simulink model "test_online"  (R2024b)
settings: Solver=FixedStepAuto  StartTime=0.0  StopTime=inf  FixedStep=0.005  RelTol=1e-3
libraries: androidsensorlib x2, deeplib x1, androidaudiovideolib x1
settings Model: Creator=alessandro  LastModifiedBy=marta
settings OptimizationCC: DefaultParameterBehavior=Inlined  EnhancedBackFolding=on  PassReuseOutputArgsAs=Individual arguments  ZeroExternalMemoryAtStartup=off  ZeroInternalMemoryAtStartup=off  MaxStackSize=64  OptimizeBlockOrder=speed  DifferentSizesBufferReuse=on  OptimizationCustomize=off  EfficientTunableParamExpr=on
settings DebuggingCC: ParameterTunabilityLossMsg=error
settings HardwareCC: ProdBitPerPointer=32  ProdBitPerSizeT=32  ProdBitPerPtrDiffT=32  ProdLargestAtomicInteger=Long  ProdLargestAtomicFloat=Double  ProdWordSize=32  ProdHWDeviceType=ARM Compatible->ARM Cortex-A (32-bit)  UseEmbeddedCoderFeatures=off  UseSimulinkCoderFeatures=off
settings SFSimCC: MATLABDynamicMemAlloc=off
settings RTWCC: Description=Embedded Coder  SystemTargetFile=ert.tlc  HardwareBoard=Android Device  TLCOptions="-aInlineSetEventsForThisBaseRateFcn=TLC_FALSE -aSuppressMultiTaskScheduler=TLC_FALSE  -aRateBasedStepFcn=0"  TemplateMakefile=ert_default_tmf  RTWVerbose=off  Toolchain=Android SDK/NDK Tools
settings CodeAppCC: ForceParamTrailComments=on  IgnoreCustomStorageClasses=off  OperatorAnnotations=on  SimulinkDataObjDesc=on  SFDataObjDesc=on  MangleLength=10  InsertBlockDesc=on
settings ERTTargetCC: SupportNonInlinedSFcns=on

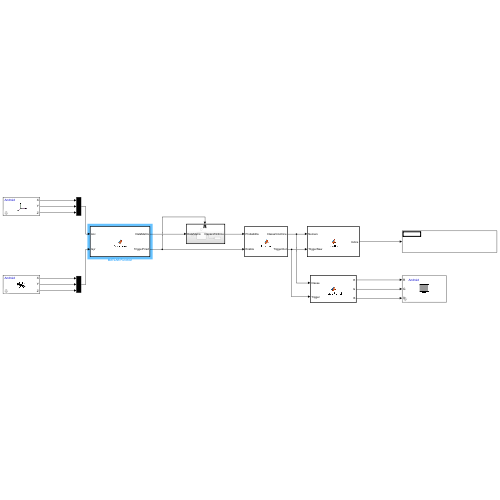
[thumbnail: Simulink's stored preview of the top-level diagram]
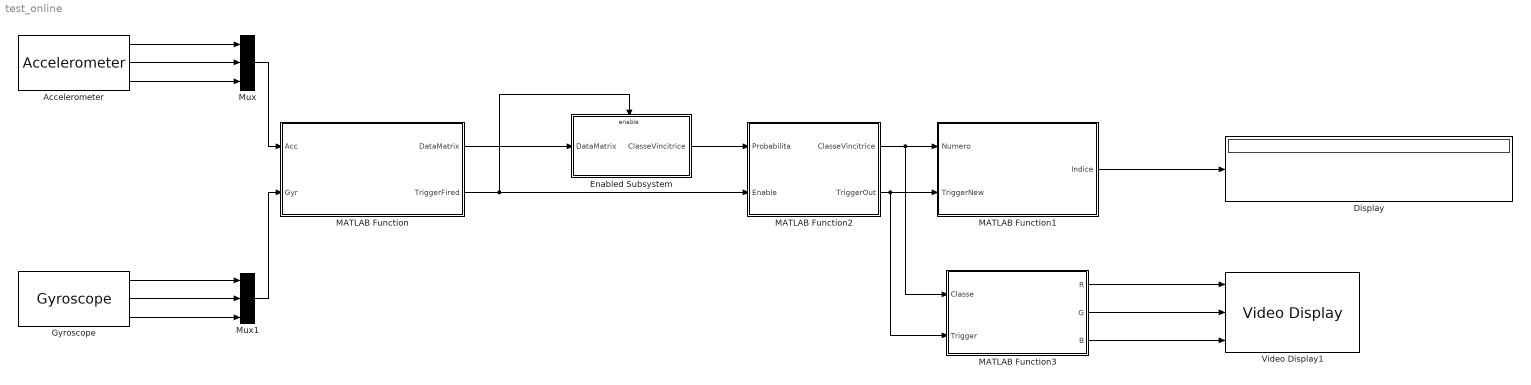
== system test_online ==
  Accelerometer : androidsensorlib/Accelerometer  OutputVector=off  SampleTime=0.005  BlockPlatform=Android
  Display : Display
  Enabled Subsystem : Subsystem  TreatAsAtomicUnit=on
  Gyroscope : androidsensorlib/Gyroscope  OutputVector=off  SampleTime=0.005  BlockPlatform=Android
  MATLAB Function : MATLAB Function  TreatAsAtomicUnit=on
  MATLAB Function1 : MATLAB Function  TreatAsAtomicUnit=on
  MATLAB Function2 : MATLAB Function  TreatAsAtomicUnit=on
  MATLAB Function3 : MATLAB Function  TreatAsAtomicUnit=on
  Mux : Mux  Inputs=3
  Mux1 : Mux  Inputs=3
  Video Display1 : androidaudiovideolib/Video Display  BlockPlatform=Android
  wires:
  MATLAB Function/1(DataMatrix) -> Enabled Subsystem/1(DataMatrix)
  MATLAB Function/2(TriggerFired) -> MATLAB Function2/2(Enable), Enabled Subsystem/Enable
  Accelerometer/1 -> Mux/1
  Accelerometer/2 -> Mux/2
  Accelerometer/3 -> Mux/3
  Mux/1 -> MATLAB Function/1(Acc)
  Gyroscope/1 -> Mux1/1
  Gyroscope/2 -> Mux1/2
  Gyroscope/3 -> Mux1/3
  Mux1/1 -> MATLAB Function/2(Gyr)
  Enabled Subsystem/1(ClasseVincitrice) -> MATLAB Function2/1(Probabilita)
  MATLAB Function2/1(ClasseVincitrice) -> MATLAB Function3/1(Classe), MATLAB Function1/1(Numero)
  MATLAB Function2/2(TriggerOut) -> MATLAB Function1/2(TriggerNew), MATLAB Function3/2(Trigger)
  MATLAB Function1/1(Indice) -> Display/1
  MATLAB Function3/1(R) -> Video Display1/1
  MATLAB Function3/2(G) -> Video Display1/2
  MATLAB Function3/3(B) -> Video Display1/3

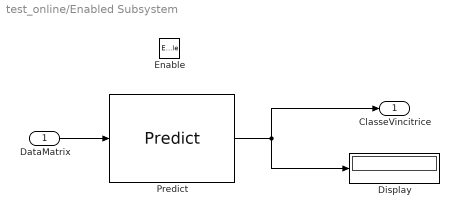
== system test_online/Enabled Subsystem ==
  DataMatrix : Inport
  Enable : EnablePort
  Display : Display
  Predict : deeplib/Predict  Network=Network from MAT-file  NetworkFunction=squeezenet  NetworkFilePath=Rete_CNN_Finale.mat  MiniBatchSize=128  InputDataFormats={ 'input', 'TCB' }  Predictions=on  Activations={}  ForceInterpretedSim=off  EnableDLNetwork=on  LastKnownNetworkFilePath='Rete_CNN_Finale.mat'  LastKnownNetworkTimeStamp=739962.956712962943129241466522216796875
  ClasseVincitrice : Outport
  wires:
  DataMatrix/1 -> Predict/1
  Predict/1 -> Display/1, ClasseVincitrice/1

== matlab function test_online/MATLAB Function ==
  data: Acc input; DataMatrix output; Gyr input; TriggerFired output
function [DataMatrix, TriggerFired] = Processor_Complete(Acc, Gyr)
    Acc = double(Acc(:)).';
    Gyr = double(Gyr(:)).';

    persistent buffer_acc buffer_gyr
    persistent state counter
    persistent baseline_ema
    persistent b_filt a_filt
    persistent z_state          
    persistent startup_timer
    persistent ema_state        

    % --- PARAMETRI ---
    FS = 200;

    WIN_LEN  = 401;
    POST_SEC = 1.0;
    SAMPLES_POST = round(POST_SEC * FS);

    WARMUP_TIME = WIN_LEN;

    % Trigger baseline EMA
    ALPHA_BASELINE = 0.01;
    K_SOGLIA = 2;
    SOGLIA_MIN = 0.1;

    % Smoothing EMA segnale
    ALPHA_SMOOTH = 0.2;

    % --- OUTPUT DEFAULT ---
    TriggerFired = false;
    DataMatrix   = zeros(WIN_LEN, 6, 'single');

    % --- INIZIALIZZAZIONE ---
    if isempty(buffer_acc)
        buffer_acc = zeros(WIN_LEN, 3);
        buffer_gyr = zeros(WIN_LEN, 3);

        state   = 0;
        counter = 0;

        baseline_ema = 0.0;
        startup_timer = WARMUP_TIME;

        [b_filt, a_filt] = butter(2, [0.5 20] / (FS/2), 'bandpass');

        nf = max(length(a_filt), length(b_filt)) - 1;
        z_state = zeros(nf, 6);

        ema_state = zeros(1, 6);
    end

    % --- COSTRUISCI CAMPIONE 1x6 ---
    raw_input = [Acc, Gyr];  % 1x6

    % --- FILTRAGGIO ONLINE CANALE-PER-CANALE ---
    filt_sample = zeros(1, 6);

    for ch = 1:6
        % filtra un campione scalare
        [y, zf] = filter(b_filt, a_filt, raw_input(ch), z_state(:,ch));
        filt_sample(ch) = y;
        z_state(:,ch) = zf;
    end

    % --- SMOOTHING EMA SUI 6 CANALI ---
    ema_state = (1 - ALPHA_SMOOTH) * ema_state + ALPHA_SMOOTH * filt_sample;
    smooth_sample = ema_state;

    Acc_Filt = smooth_sample(1:3);
    Gyr_Filt = smooth_sample(4:6);

    % --- AGGIORNAMENTO BUFFER ---
    buffer_acc = [buffer_acc(2:end, :); Acc_Filt];
    buffer_gyr = [buffer_gyr(2:end, :); Gyr_Filt];

    % --- WARMUP (aggiorna baseline) ---
    acc_y = abs(Acc_Filt(2));

    if startup_timer > 0
        baseline_ema = (1 - ALPHA_BASELINE) * baseline_ema + ALPHA_BASELINE * acc_y;
        startup_timer = startup_timer - 1;
        return;
    end

    % --- SOGLIA ADATTIVA ---
    baseline_ema = (1 - ALPHA_BASELINE) * baseline_ema + ALPHA_BASELINE * acc_y;
    soglia = K_SOGLIA * baseline_ema;
    if soglia < SOGLIA_MIN
        soglia = SOGLIA_MIN;
    end

    % --- MACCHINA A STATI ---
    if state == 0
        if acc_y > soglia
            state = 1;
            counter = 0;
        end

    else % state == 1
        counter = counter + 1;

        if counter >= SAMPLES_POST
            % --- Z-SCORE SU FINESTRA ---
            mu_a  = mean(buffer_acc, 1);
            sig_a = std(buffer_acc, 0, 1);
            mu_g  = mean(buffer_gyr, 1);
            sig_g = std(buffer_gyr, 0, 1);

            sig_a(sig_a == 0) = 1;
            sig_g(sig_g == 0) = 1;

            a_norm = (buffer_acc - mu_a) ./ sig_a;
            g_norm = (buffer_gyr - mu_g) ./ sig_g;

            DataMatrix   = single([a_norm, g_norm]);
            TriggerFired = true;

            state = 0;
            counter = 0;
        end
    end
end

== matlab function test_online/MATLAB Function2 ==
  data: Probabilita input; ClasseVincitrice output; Enable input; TriggerOut output
function [ClasseVincitrice, TriggerOut] = Decisore(Probabilita, Enable)
    % INPUT: 
    % - Probabilita: vettore uscita dalla rete
    % - Enable: il segnale 'TriggerFired' che esce dal blocco Processor

    SOGLIA = 0.80; 

    % Se il Processor dice che NON c'è un nuovo pugno (Enable=0),
    % ignoriamo completamente cosa dice la rete (che potrebbe essere bloccata a 1).
    if Enable == 0
        ClasseVincitrice = 0; % Riposo forzato
        TriggerOut = 0;
        return; % Usciamo subito
    end

    % --- Se siamo qui, il Trigger è ATTIVO, analizziamo le probabilità ---
    if Probabilita(1) > SOGLIA
        ClasseVincitrice = 1; % JAB
        TriggerOut = 1;      
    elseif Probabilita(2) > SOGLIA
        ClasseVincitrice = 2; % MONTANTE
        TriggerOut = 1;       
    else
        ClasseVincitrice = 0; 
        TriggerOut = 0;
    end
end

== matlab function test_online/MATLAB Function1 ==
  data: Numero input; Indice output; TriggerNew input
function Indice = Traduttore(Numero, TriggerNew)
    % Output: 0, 1, 2 (Numeri interi)
    % NON usare stringhe qui dentro!
    
    persistent Timer ValoreSalvato
    DURATA_SCRITTA = 600; 
    
    if isempty(Timer)
        Timer = 0;
        ValoreSalvato = 0;
    end
    
    Num = double(Numero);
    Trig = double(TriggerNew);
    
    if Trig > 0
        ValoreSalvato = Num;
        Timer = DURATA_SCRITTA;
    end
    
    if Timer > 0
        Timer = Timer - 1;
        Indice = ValoreSalvato;
    else
        Indice = 0; 
    end
end

== matlab function test_online/MATLAB Function3 ==
  data: Classe input; R output uint8 size=[640 480]; G output uint8 size=[640 480]; B output uint8 size=[640 480]; Trigger input
function [R, G, B] = ImagePanel(Classe, Trigger)
    % INPUT: Classe (0,1,2), Trigger (0,1)
    % OUTPUT: Matrici Sicure 640x480
    
    persistent R_Jab G_Jab B_Jab
    persistent R_Mont G_Mont B_Mont
    persistent R_Fermo G_Fermo B_Fermo
    persistent Timer ClasseBloccata
    
    % --- NUOVE DIMENSIONI SICURE ---
    H = 640; % Altezza
    W = 480; % Larghezza
    HOLD_TIME = 200; 
    
    % --- INIZIALIZZAZIONE ---
    if isempty(R_Jab)
        Timer = 0;
        ClasseBloccata = 0;
        
        % Pre-allocazione
        Dummy = zeros(H, W, 'uint8');
        R_Jab=Dummy; G_Jab=Dummy; B_Jab=Dummy;
        R_Mont=Dummy; G_Mont=Dummy; B_Mont=Dummy;
        R_Fermo=Dummy; G_Fermo=Dummy; B_Fermo=Dummy;

        % Caricamento
        Pack = coder.load('dati.mat');
        
        % ESTRAZIONE (Taglio sicuro)
        RawJ = Pack.J;
        R_Jab = RawJ(1:H, 1:W, 1); G_Jab = RawJ(1:H, 1:W, 2); B_Jab = RawJ(1:H, 1:W, 3);
        
        RawM = Pack.M;
        R_Mont = RawM(1:H, 1:W, 1); G_Mont = RawM(1:H, 1:W, 2); B_Mont = RawM(1:H, 1:W, 3);
        
        RawF = Pack.F;
        R_Fermo = RawF(1:H, 1:W, 1); G_Fermo = RawF(1:H, 1:W, 2); B_Fermo = RawF(1:H, 1:W, 3);
    end
    
    % --- LOGICA TRIGGER (Resto invariato) ---
    ClasseIn = double(Classe);
    if Trigger > 0 && ClasseIn > 0
        ClasseBloccata = ClasseIn;
        Timer = HOLD_TIME;
    end
    
    if Timer > 0
        Timer = Timer - 1;
        Show = ClasseBloccata;
    else
        Show = 0; 
    end
    
    % --- OUTPUT ---
    if Show == 1
        R = R_Jab; G = G_Jab; B = B_Jab;
    elseif Show == 2
        R = R_Mont; G = G_Mont; B = B_Mont;
    else
        R = R_Fermo; G = G_Fermo; B = B_Fermo;
    end
end
